simulink model "nonlinear_model"  (R2023b)
settings: Solver=VariableStepAuto  StartTime=0.0  StopTime=10.0  RelTol=1e-3
libraries: slpidlib x1, simulink_extras x1
settings Model: Creator=USER  LastModifiedBy=USER

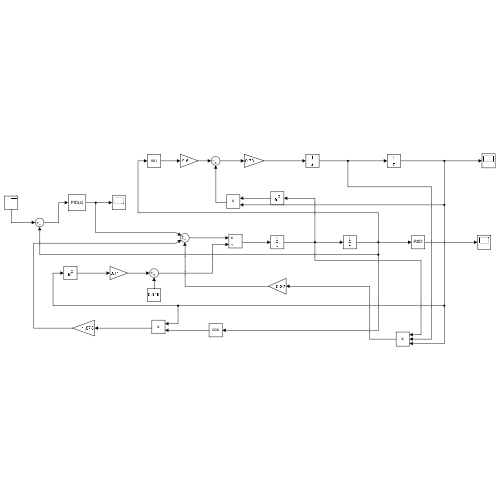
[thumbnail: Simulink's stored preview of the top-level diagram]
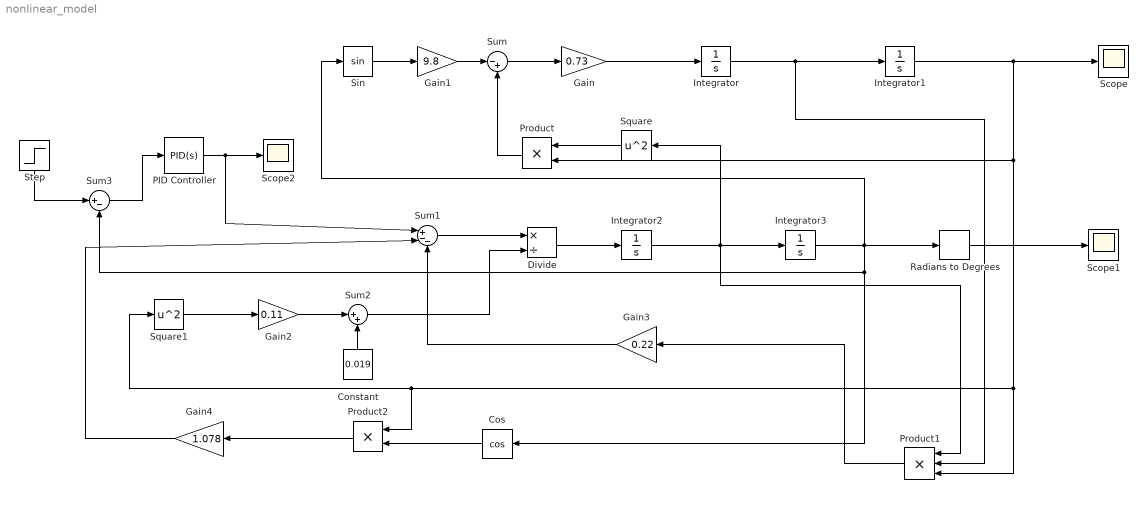
== system nonlinear_model ==
  Constant : Constant  Value=0.019
  Cos : Trigonometry  Operator=cos
  Divide : Product  Inputs=*/
  Gain : Gain  Gain=0.73
  Gain1 : Gain  Gain=9.8
  Gain2 : Gain  Gain=0.11
  Gain3 : Gain  Gain=0.22
  Gain4 : Gain  Gain=1.078
  Integrator{,1..3} (4 alike) : Integrator
  PID Controller : slpidlib/PID Controller  Controller=PID  Form=Parallel  TimeDomain=Continuous-time  UseExternalTs=off  SampleTime=-1  IntegratorMethod=Forward Euler  FilterMethod=Forward Euler  ControllerParametersSource=internal  P=10  I=8  UseKiTs=off  D=10  N=1  UseFilter=on  TunerSelectOption=Transfer Function Based (PID Tuner App)  InitialConditionSource=internal  InitialConditionForIntegrator=0  InitialConditionForFilter=0  DifferentiatorICPrevScaledInput=0  ExternalReset=none  TrackingMode=off  Kt=1  LimitOutput=off  SatLimitsSource=internal  UpperSaturationLimit=inf  LowerSaturationLimit=-inf  LinearizeAsGain=on  AntiWindupMode=none  Kb=1  LimitIntegrator=off  UpperIntegratorSaturationLimit=inf  LowerIntegratorSaturationLimit=-inf  POutMin=[]  POutMax=[]  IOutMin=[]  IOutMax=[]  DOutMin=[]  DOutMax=[]  NOutMin=[]  NOutMax=[]  SumOutMin=[]  SumOutMax=[]  SaturationOutMin=[]  SaturationOutMax=[]  PParamMin=[]  PParamMax=[]  IParamMin=[]  IParamMax=[]  DParamMin=[]  DParamMax=[]  NParamMin=[]  NParamMax=[]  KbParamMin=[]  KbParamMax=[]  KtParamMin=[]  KtParamMax=[]  KbOutMin=[]  KbOutMax=[]  KtOutMin=[]  KtOutMax=[]  IntegratorOutMin=[]  IntegratorOutMax=[]  FilterOutMin=[]  FilterOutMax=[]  SumI1OutMin=[]  SumI1OutMax=[]  SumI2OutMin=[]  SumI2OutMax=[]  SumI3OutMin=[]  SumI3OutMax=[]  SumI4OutMin=[]  SumI4OutMax=[]  SumDOutMin=[]  SumDOutMax=[]  DifferentiatorOutMin=[]  DifferentiatorOutMax=[]  FilterDiffOutCoefMin=[]  FilterDiffOutCoefMax=[]  ReciprocalOutMin=[]  ReciprocalOutMax=[]  SumDenOutMin=[]  SumDenOutMax=[]  SumNumOutMin=[]  SumNumOutMax=[]  DivideOutMin=[]  DivideOutMax=[]  UdiffTsProdOutMin=[]  UdiffTsProdOutMax=[]  NTsProdOutMin=[]  NTsProdOutMax=[]  UintegralTsProdOutMin=[]  UintegralTsProdOutMax=[]  UngainTsProdOutMin=[]  UngainTsProdOutMax=[]  ClampingZeroOutDataTypeStr=Inherit: Inherit via back propagation  ClampingZeroOutMin=[]  ClampingZeroOutMax=[]  FilterDenConstantOutDataTypeStr=Inherit: Inherit via back propagation  FilterDenConstantOutMin=[]  FilterDenConstantOutMax=[]  PCopyOutDataTypeStr=Inherit: Inherit via back propagation  PCopyOutMin=[]  PCopyOutMax=[]  NCopyOutDataTypeStr=Inherit: Inherit via back propagation  NCopyOutMin=[]  NCopyOutMax=[]  IntegratorContinuousStateAttributes=''  IntegratorStateMustResolveToSignalObject=off  IntegratorRTWStateStorageClass=Auto  FilterContinuousStateAttributes=''  FilterStateMustResolveToSignalObject=off  FilterRTWStateStorageClass=Auto  ParallelPVariant=InternalParameters  IdealPVariant=Disabled  IVariant=InternalParameters  DVariant=InternalParameters  IntegratorVariant=Continuous  SatVariant=Disabled  AWVariant=Passthrough  PCopyVariant=Disabled  TRVariant=Disabled  FdbkBlocksVariant=Forward  IdealPFdbkVariant=Disabled  SatFdbkVariant=Disabled  DerivativeFilterVariant=ContFilter  NVariant=InternalParameters  NCopyVariant=Disabled  FilterICVariant=InternalICsFilter  IntegratorICVariant=InternalICs  ExternalResetVariant=Disabled  TRSumVariant=Passthrough  SumFdbkVariant=Disabled  SumVariant=Sum_PID  TsampFilterVariant=InternalTs  TsampNgainVariant=Passthrough  TsampIntegralVariant=Disabled_SignalSpec  ExternalSaturationOutDataTypeStr=Inherit: Same as second input
  Product : Product
  Product1 : Product  Inputs=3
  Product2 : Product
  Radians to Degrees : simulink_extras/Transformations/Radians to Degrees
  Scope : Scope
  Scope1 : Scope
  Scope2 : Scope
  Sin : Trigonometry
  Square : Math  Operator=square
  Square1 : Math  Operator=square
  Step : Step  After=10*pi/180  SampleTime=0
  Sum : Sum  Inputs=|-+
  Sum1 : Sum  Inputs=|+--
  Sum2 : Sum  Inputs=|++
  Sum3 : Sum  Inputs=|+-
  wires:
  Gain/1 -> Integrator/1
  Sum/1 -> Gain/1
  Gain1/1 -> Sum/1
  Sin/1 -> Gain1/1
  Square/1 -> Product/1
  Sum1/1 -> Divide/1
  Divide/1 -> Integrator2/1
  Integrator2/1 -> Square/1, Integrator3/1, Product1/1
  Integrator3/1 -> Sum3/2, Cos/1, Radians to Degrees/1, Sin/1
  Gain2/1 -> Sum2/1
  Square1/1 -> Gain2/1
  Constant/1 -> Sum2/2
  Sum2/1 -> Divide/2
  Gain3/1 -> Sum1/3
  Product2/1 -> Gain4/1
  Gain4/1 -> Sum1/2
  Cos/1 -> Product2/2
  Product1/1 -> Gain3/1
  Product/1 -> Sum/2
  Step/1 -> Sum3/1
  PID Controller/1 -> Sum1/1, Scope2/1
  Sum3/1 -> PID Controller/1
  Radians to Degrees/1 -> Scope1/1
  Integrator1/1 -> Scope/1, Product/2, Product1/3, Square1/1, Product2/1
  Integrator/1 -> Integrator1/1, Product1/2
